simulink library "AFCToolbox"  (R2025b)
settings: Solver=VariableStepAuto  StartTime=0.0  StopTime=10.0  RelTol=1e-3
undefined symbols (not defined in the file or in its folder): AFC5Toolbox_SimuMoudle, ax, ay, az, C_d, C_dm, C_m, C_t, Control, d, declination_table, dp0, dp1, dp2, dp3, dt, euler_0, g0, I_xyz, inclination_table, J_m, lmd_high, lmd_low, lp_acc_knoise, lp_acc_max, lp_acc_min, lp_acc_seed, lp_GPS_BL_max, lp_GPS_BL_min, lp_GPS_H_max, lp_GPS_H_min, lp_GPS_knoise, lp_GPS_seed, lp_GPS_vel_max, lp_GPS_vel_min, lp_gyro_knoise, lp_gyro_max, lp_gyro_min, lp_gyro_seed, lp_hf_vwind, lp_hs_vwind_interp, lp_kaerorho, lp_kaeroT, lp_kIxyz, lp_kmass, lp_momentx_A0, lp_momentx_Af, lp_momentx_ts, lp_momenty_A0, lp_momenty_Af, lp_momenty_ts, lp_momentz_A0, lp_momentz_Af, lp_momentz_ts, lp_vf_vwind, lp_vs_vwind_interp, lp_vwind_thetax, lp_vwind_thetaz, mass, MB_states ... (+52)
libraries: $bdroot x104, simulink x75, etargetslib x32, sharedtransform x13, simulink_extras x12, dspstat3 x11, aerolibconvert2 x9, aerolibtransform2 x3, aerolibutil x2, matrix_library x1
(part 11 of 11)

== matlab function AFCToolbox/基础导航算法模型库/ECL EKF/init_state/InitState_baro1/TD_baro/MATLAB Function2 ==
  data: T input single; u1 output; u0 input; u1 input single; u2 input single; h input single; r input single; u2 output
function [u1,u2]=diff_TD_2(T,u0,u1,u2,h,r)
    %init
    %T是信号周期，u0原始信号输入，u1跟踪原始信号，u2原始信号差分值，
    %h滤波因子（h=T时接近一阶差分）越大滤波好延迟大；r速度因子，越大跟踪的越快但是噪声放大；

x1=0; x2=0;
delta=0;
delta0=0;
y=0;
fabs_y=0;
a0=0;
a=0;
fst=0;

x1 = u1;
x2 = u2;
delta = r*h;
delta0 = delta*h;
y = x1 - u0 + h*x2;
fabs_y = abs(y);   
a0 = sqrt(delta*delta + 8 * r*fabs_y);

if (fabs_y <= delta0)
	a = x2 + y / h;
else
    a = x2 + 0.5*(a0 - delta)*sign(y);
end

if (abs(a) <= delta)
	fst = -r*a / delta;
else
	fst = -r*sign(a);
end
u1 = single(x1 + T*x2); %计算跟踪信号
u2 = single(x2 + T*fst); % 计算微分信号

== matlab function AFCToolbox/基础导航算法模型库/ECL EKF/init_state/InitState_baro1/compensateBaroForDynamicPressure ==
  data: baro_alt_uncompensated input; baro_sample_new output; output_quaternion input; output_new_vel input; state_wind_vel input; delta_ang input
function baro_sample_new  = compensateBaroForDynamicPressure(baro_alt_uncompensated,...
    output_quaternion,...
    output_new_vel,...
    state_wind_vel,...    %filter output on the non-delayed time horizon
    delta_ang) %delta angle in body frame (integrated gyro measurements) (rad)
    
% EKF2.cpp -> UpdateBaroSample(...) ->
% ~ estimator_interface.cpp -> setBaroData(...) ->
% ~ ekf_helper.cpp -> compensateBaroForDynamicPressure(...)

dt = 0.01;
CONSTANTS_ONE_G = 9.80665;
CONSTANTS_AIR_DENSITY_SEA_LEVEL_15C = 1.225; % air density (kg/m**3)
air_density = CONSTANTS_AIR_DENSITY_SEA_LEVEL_15C;

params.static_pressure_coef_xp = 1;
params.static_pressure_coef_yp = -1;

params.static_pressure_coef_xn = 0;
params.static_pressure_coef_yn = 0;

params.static_pressure_coef_z = 0;

params.max_correction_airspeed = 20;
params.imu_pos_body = zeros(1,3);  % xyz position of IMU in body frame (m)

% calculate static pressure error = Pmeas - Ptruth
R_to_body = transpose(Quat2Tbn(normQuat(output_quaternion)));

% Calculate airspeed in body frame
ang_rate = delta_ang / dt;
% vel_imu_rel_body_ned = cross(ang_rate,params.imu_pos_body);
% vel_imu_rel_body_ned = Quat2Tbn(normQuat(output_quaternion))*vel_imu_rel_body_ned;
vel_imu_rel_body_ned = [0;0;0];

velocity_earth = output_new_vel - vel_imu_rel_body_ned;

wind_velocity_earth = [state_wind_vel(1), state_wind_vel(2), 0.0];

airspeed_earth = velocity_earth - wind_velocity_earth;

airspeed_body = R_to_body * airspeed_earth;

K_pstatic_coef = zeros(3,1);
if airspeed_body(1) > 0
    K_pstatic_coef(1) = params.static_pressure_coef_xp;
else
    K_pstatic_coef(1) = params.static_pressure_coef_xn;
end
if airspeed_body(2) > 0
    K_pstatic_coef(2) = params.static_pressure_coef_yp;
else
    K_pstatic_coef(2) = params.static_pressure_coef_yn;
end
K_pstatic_coef(3) = params.static_pressure_coef_z;
airspeed_squared = zeros(1,3);
K = emult(airspeed_body);
for i = 1:3
    airspeed_squared(i) = min(K(i), power((params.max_correction_airspeed),2));
end
pstatic_err = 0.5 * air_density * (airspeed_squared*(K_pstatic_coef));

% correct baro measurement using pressure error estimate and assuming sea level gravity
baro_sample_new = baro_alt_uncompensated + pstatic_err / (air_density * CONSTANTS_ONE_G);

== matlab function AFCToolbox/基础导航算法模型库/ECL EKF/init_state/LLA2NED/initGPSLLA ==
  data: QGCinitflag input; gpsLLA0_rad output; GPSfixtype input; gps_LLA_rad input; init_GPSLLAflag output
function [gpsLLA0_rad,init_GPSLLAflag] = initGPSLLA0(QGCinitflag,GPSfixtype,gps_LLA_rad)
    persistent initGPSLLAflag;
    persistent gpsLLA0;

    if isempty(initGPSLLAflag)
        initGPSLLAflag = 0;
    end
    if isempty(gpsLLA0)
        % 初始GPS未进入定位状态，给定值
        % gpsLLA0 = [28.2/57.3;113/57.3;0];
        gpsLLA0 = zeros(3,1);
    end
    if (initGPSLLAflag == 0 && GPSfixtype >= 1) || (QGCinitflag == 1 && GPSfixtype >= 1)
        % 当GPS第一次初始化位置时，当GPSfixtype >=1 时，自动初始化一次位置，initGPSLLAflag置1
        % 或者是利用QGCinitflag地面站重新修正，不过需要满足GPSfixtype>=1的条件
        gpsLLA0 = gps_LLA_rad;
        initGPSLLAflag = 1;
    end
    gpsLLA0_rad = gpsLLA0;
    init_GPSLLAflag = initGPSLLAflag;
end

== matlab function AFCToolbox/基础导航算法模型库/ECL EKF/init_state/MATLAB Function1 ==
  data: yaw output; quat input; quat output; magMea input; declination input; euler output
function [yaw,quat,euler] = AlignHeading( ...
    quat, ... % quaternion state vector
    magMea, ... % body frame magnetic flux measurements 
    declination)  % Estimated magnetic field delination at current location (rad)

% Get the Euler angles and set yaw to zero
euler = QuatToEul(quat);
euler(3) = 0;

% calculate the rotation matrix from body to earth frame,N→B
quat_zero_yaw = EulToQuat(euler);
Tbn_zero_yaw = Quat2Tbn(quat_zero_yaw);

% Rotate the magnetic field measurement into earth frame,                  mb1=Rbn*mb
magMeasNED = Tbn_zero_yaw*magMea;

% Use the projection onto the horizontal to calculate the yaw angle,       φ=-atan2（mb1y,mb1x）
euler(3) = declination - atan2(magMeasNED(2),magMeasNED(1));
yaw = -atan2(magMeasNED(2),magMeasNED(1));
%euler(3) = -45/57.3;
% convert to a quaternion
quat = EulToQuat(euler);

end

== matlab function AFCToolbox/基础导航算法模型库/ECL EKF/init_state/State_mag1/Subsystem1/Subsystem/MATLAB Function1 ==
  data: lon input; Lon output
function Lon = limit(lon)
SAMPLING_MAX_LON = 180;
SAMPLING_MIN_LON = -180;
if (lon > SAMPLING_MAX_LON)
		Lon = lon - 360;
elseif (lon < SAMPLING_MIN_LON) 
	Lon = lon + 360;
else
    Lon = lon;
end

== matlab function AFCToolbox/基础导航算法模型库/ECL EKF/init_state/State_mag1/Subsystem1/Subsystem2/MATLAB Function1 ==
  data: lon input; Lon output
function Lon = limit(lon)
SAMPLING_MAX_LON = 180;
SAMPLING_MIN_LON = -180;
if (lon > SAMPLING_MAX_LON)
		Lon = lon - 360;
elseif (lon < SAMPLING_MIN_LON) 
	Lon = lon + 360;
else
    Lon = lon;
end

== matlab function AFCToolbox/基础导航算法模型库/ECL EKF/init_state/State_mag1/Subsystem1/Subsystem3/MATLAB Function1 ==
  data: lon input; Lon output
function Lon = limit(lon)
SAMPLING_MAX_LON = 180;
SAMPLING_MIN_LON = -180;
if (lon > SAMPLING_MAX_LON)
		Lon = lon - 360;
elseif (lon < SAMPLING_MIN_LON) 
	Lon = lon + 360;
else
    Lon = lon;
end

== stateflow chart AFCToolbox/SimuMoudle/Equations of Motion1/Chart ==
  state Land
    en, du: ground_contact = 1;
  state Flight
    en, du: ground_contact = 0;
  (default) -> Land
  Flight -> Land : [h<=0 && vel(3) >0]
  Land -> Flight : [acc(3)<0]
  data: h input; vel input; acc input; ground_contact output

== matlab function AFCToolbox/基础导航算法模型库/ECL EKF/init_state/State_mag1/initMag1 ==
  data: GPSfixtype input; init_mag output; mag input; init_magflag output
function [init_mag,init_magflag] = initMag(GPSfixtype,mag)
    persistent initMAGflag;
    persistent initmag;

    if isempty(initMAGflag)
        initMAGflag = 0;
    end
    if isempty(initmag)
        % 初始GPS未进入定位状态，给定值
        initmag = zeros(3,1);
 
    end
    if (initMAGflag == 0 && GPSfixtype >= 1) 
        % 当GPS第一次初始化位置时，当GPSfixtype >=1 时，自动初始化一次位置，initGPSLLAflag置1
        % 或者是利用QGCinitflag地面站重新修正，不过需要满足GPSfixtype>=1的条件
        initmag = mag;       
        initMAGflag = 1;
    end
    init_mag = initmag;
    init_magflag = initMAGflag;
end

== matlab function AFCToolbox/基础导航算法模型库/ECL EKF/Subsystem/GPS Fusion1/Control BARO_Hgt Fusion/Control Baro_Height Fusion1 ==
  data: states input; states output; P input; measHgt input; P output; innovation output; innov_var output; baro_b_est_getBias input; baro_hgt_offset input; params_baro_noise input
function [...
    states, ... % state vector after fusion of measurements
    P, ... % state covariance matrix after fusion of corrections
    innovation,... % D position innovations (m)
    innov_var] ... % D position innovation variance (m^2)
    = FusePosition( ...
    states, ... % predicted states from the INS
    P, ... % predicted covariance
    measHgt,... % D position measurements form baro (m)
    baro_b_est_getBias,...%Baro bias estimation using GPS altitude
    baro_hgt_offset,...%baro height reading at the local NED origin (m)
params_baro_noise)
% ~ control.cpp -> controlHeightFusion() -> updateBaroHgt() -> fuseBaroHgt()

% innovation gate size
% barometric and GPS height innovation consistency gate size (STD)
params.baro_innov_gate = 5; 
innov_gate = max(params.baro_innov_gate, 1);
% observation noise for barometric height fusion (m),RBaro
% params_baro_noise = 0.25; 
obs_var = power(max(params_baro_noise, 0.1),2);

%% barohgt fusion
H = zeros(1,24);
Kfusion = zeros(24,1);
KHP = zeros(24,24);
% position states start at index 10
stateIndex = 10;
% Calculate the observation Jacobian
% H_Baro is 1
H(stateIndex) = 1;

% Calculate the residual covarianc                    S = (HBaro * Pk+1|k * HGPS_T) + RBaro
innov_var = H*P*transpose(H) + obs_var;

% Calculate the velocity measurement innovation,where yk = zBaro + HBaro * Xk+1|k  
% Calculate the vertical position height innovation (posD is opposite sign to height
measHgt = measHgt - baro_b_est_getBias - baro_hgt_offset;
innovation = measHgt + states(stateIndex);

%% set Estimator Aid Status Test Ratio
% Apply an innovation consistency check
if (innovation^2 / (innov_gate^2 * innov_var)) > 1.0
    return;
end
    
%% Calculate Kalman gains and update states and covariances
%calculate kalman gain K = P*HT*S, where S = innov_var and HBaro = eyes(1:2,8:9)
for  row = 1:24
    state_index = 10;
    Kfusion(row) = P(row, state_index) / innov_var;
end
% Calculate state corrections                       K_yk = K*yk
K_yk = Kfusion * innovation;
% Apply the state corrections                       Xk+1|k+1 = Xk+1|k + K_yk
states = states - K_yk;
% caculate intermediate KHP                         KHP = K * HBaro * Pk+1|k
for row = 1:24
    for column = 1:24
        KHP(row, column) = Kfusion(row) * P(state_index, column);
    end
end
% Update the covariance P                           Pk+1|k+1 = [I − K * HGPS] * Pk+1|k
P = P - KHP;
%% Force symmetry on the covariance matrix to prevent ill-conditioning
P = 0.5*(P + transpose(P));
% ensure diagonals are positive
for i=1:24
    if P(i,i) < 0
        P(i,i) = 0;
    end
end
end

== matlab function AFCToolbox/基础导航算法模型库/ECL EKF/Subsystem/GPS Fusion1/Control GPS_Pos Fusion1 ==
  data: states input; states output; P input; measPos input; innov_gate input; obs_var input; P output; innovation output; innov_var output; contrl_GPSflag input; gps_alt_ref input; gps_hgt_offset input
function [...
    states, ... % state vector after fusion of measurements
    P, ... % state covariance matrix after fusion of corrections
    innovation,... % NE position innovations (m)
    innov_var] ... % NE position innovation variance (m^2)
    = FusePosition( ...
    states, ... % state vector after fusion of measurements
    P, ... % state covariance matrix after fusion of corrections
    measPos, ... % NED position measurements (m)
    innov_gate, ... % Size of the innovation consistency check gate (std-dev)
    obs_var,... % position observation variance (m)^2
    contrl_GPSflag,...
    gps_alt_ref,...
    gps_hgt_offset)
%% x&y position
innovation = zeros(1,3);
H = zeros(3,24);
innov_var = zeros(1,3);
Kfusion = zeros(24,3);
KHP = zeros(24,24);

for obs_index = 1:2
   % position states start at index 8
   stateIndex = 7 + obs_index;
   % Calculate the observation Jacobian
   % H_GPS is eyes(1:2,8:9)
   H(obs_index,stateIndex) = 1;
   % Calculate the residual covarianc                    S = (HGPS * Pk+1|k * HGPS_T) + RGPS
   innov_var(obs_index) = P(7 + obs_index, 7 + obs_index) + obs_var(obs_index);
   % Calculate the velocity measurement innovation,where yk = HGPS * Xk+1|k - zGPS
   innovation(obs_index) =  states(stateIndex) - measPos(obs_index);
end

%% set Estimator Aid Status Test Ratio
% Apply an innovation consistency check
for obs_index = 1:2
    if (innovation(obs_index)^2 / (innov_gate^2 * innov_var(obs_index))) > 1.0
        return;
    end
    
end

%% Calculate Kalman gains and update states and covariances
%calculate kalman gain K = PHS, where S = innov_var and HGPS = eyes(1:2,8:9)
for obs_index = 1:2
    for  row = 1:24
        state_index = obs_index + 7;
	    Kfusion(row,obs_index) = P(row, state_index) / innov_var(obs_index);
    end
    % Calculate state corrections                       K_yk = K*yk
    K_yk = Kfusion(:,obs_index) * innovation(obs_index);
    % Apply the state corrections                       Xk+1|k+1 = Xk+1|k - K_yk
    states = states - K_yk;
    % caculate intermediate KHP                         KHP = K * HGPS * Pk+1|k
    for row = 1:24
        for column = 1:24
            KHP(row, column) = Kfusion(row,obs_index) * P(state_index, column);
        end
    end
    % Update the covariance P                           Pk+1|k+1 = [I − K * HGPS] * Pk+1|k
    P = P - KHP;
    % Force symmetry on the covariance matrix to prevent ill-conditioning
    P = 0.5*(P + transpose(P));
    % ensure diagonals are positive
    for i=1:24
        if P(i,i) < 0
            P(i,i) = 0;
        end
    end
end

%% z position
if contrl_GPSflag == 1
    obs_index = 3;
    % position states start at index 8
    stateIndex = 10;
    % Calculate the observation Jacobian
    % H_GPS is eyes(1:2,8:9)
    H(obs_index,stateIndex) = 1;
    % Calculate the residual covarianc                    S = (HGPS * Pk+1|k * HGPS_T) + RGPS
    innov_var(obs_index) = P(7 + obs_index, 7 + obs_index) + obs_var(obs_index);
    % Calculate the velocity measurement innovation,where yk =  HGPS * Xk+1|k - zGPS  
     measPos(obs_index) = -(measPos(obs_index) - gps_alt_ref - gps_hgt_offset);
    innovation(obs_index) = states(stateIndex) - measPos(obs_index);

    %% set Estimator Aid Status Test Ratio
    % Apply an innovation consistency check
    if (innovation(obs_index)^2 / (innov_gate^2 * innov_var(obs_index))) > 1.0
        return;
    end

    %% Calculate Kalman gains and update states and covariances
    %calculate kalman gain K = PHS, where S = innov_var and HGPS = eyes(1:2,8:9)
    for  row = 1:24
        state_index = 10;
	    Kfusion(row,obs_index) = P(row, state_index) / innov_var(obs_index);
    end
    % Calculate state corrections                       K_yk = K*yk
    K_yk = Kfusion(:,obs_index) * innovation(obs_index);
    % Apply the state corrections                       Xk+1|k+1 = Xk+1|k - K_yk
    states = states - K_yk;
    % caculate intermediate KHP                         KHP = K * HGPS * Pk+1|k
    for row = 1:24
        for column = 1:24
            KHP(row, column) = Kfusion(row,obs_index) * P(state_index, column);
        end
    end
    % Update the covariance P                           Pk+1|k+1 = [I − K * HGPS] * Pk+1|k
    P = P - KHP;
    % Force symmetry on the covariance matrix to prevent ill-conditioning
    P = 0.5*(P + transpose(P));
    % ensure diagonals are positive
    for i=1:24
        if P(i,i) < 0
            P(i,i) = 0;
        end
    end
end
end

== matlab function AFCToolbox/基础导航算法模型库/ECL EKF/Subsystem/GPS Fusion1/Control GPS_Vel Fusion1 ==
  data: states input; states output; P input; measVel input; innov_gate input; obs_var input; P output; innovation output; innov_var output
function [...
    states, ... % state vector after fusion of measurements
    P, ... % state covariance matrix after fusion of corrections
    innovation,... % NED velocity innovations (m/s)
    innov_var] ... % NED velocity innovation variance ((m/s)^2)
    = FuseVelocity( ...
    states, ... % state vector after fusion of measurements
    P, ... % state covariance matrix after fusion of corrections
    measVel, ... % NED velocity measurements (m/s)
    innov_gate, ... % Size of the innovation consistency check gate (std-dev)
    obs_var) % velocity observation variance (m/s)^2



%% vel
innovation = zeros(1,3);
innov_var = zeros(1,3);
H = zeros(3,24);
Kfusion = zeros(24,3);
KHP = zeros(24,24);

for obs_index = 1:3
   % velocity states start at index 5
   state_index = obs_index + 4;
   % Calculate the observation Jacobian
   % H_GPS is eyes(1:3,5:8)
   H(obs_index,state_index) = 1;
   % S = (HGPS * Pk+1|k * HGPS_T) + RGPS
   innov_var(obs_index) = P(4 + obs_index, 4 + obs_index) + obs_var(obs_index);
   % Calculate the velocity measurement innovation,where yk =  HGPS * Xk+1|k - zGPS  
   innovation(obs_index) = states(state_index) - measVel(obs_index);
end

%% set Estimator Aid Status Test Ratio
% Apply an innovation consistency check
for obs_index = 1:3
    if (innovation(obs_index)^2 / (innov_gate^2 * innov_var(obs_index))) > 1.0
        return;
    end
    
end

%% Calculate Kalman gains and update states and covariances
%calculate kalman gain K = PHS, where S = innov_var and HGPS = eyes(1:3,5:8)
for obs_index = 1:3
    for  row = 1:24
        state_index = obs_index + 4;
	    Kfusion(row,obs_index) = P(row, state_index) / innov_var(obs_index);
    end
    % Calculate state corrections K_yk = K*yk
    K_yk = Kfusion(:,obs_index) * innovation(obs_index);
    % Apply the state corrections Xk+1|k+1 = Xk+1|k - K_yk
    states = states - K_yk;
    % KHP = K * HGPS * Pk+1|k
    for row = 1:24
        for column = 1:24
            KHP(row, column) = Kfusion(row,obs_index) * P(state_index, column);
        end
    end
    % Pk+1|k+1 = [I − K * HGPS] * Pk+1|k
    P = P - KHP;
    % Force symmetry on the covariance matrix to prevent ill-conditioning
    P = 0.5*(P + transpose(P));
    % ensure diagonals are positive
    for i=1:24
        if P(i,i) < 0
            P(i,i) = 0;
        end
    end
end
